simulink model "Generator_Testrig"  (R2025a)
settings: Solver=ode23t  StartTime=0.0  StopTime=15  MaxStep=0.01  RelTol=1e-5  EnableMultiTasking=on
PreLoadFcn:
  | load Generator_Test_DATA
PostLoadFcn:
  | warning off ne_sli:simulator:input:FilteredInputs
undefined symbols (not defined in the file or in its folder): radps2rpm
libraries: fl_lib x6, nesl_utility x4, Generator_Lib x3, Geartrain_Lib x1, simulink x1
Description:
  | Copyright 2009-2024 The MathWorks, Inc. MathWorks, Inc.
settings Model: Creator=smiller  LastModifiedBy=smiller
settings SolverCC: AlgebraicLoopSolver=TrustRegion
settings DataIOCC: LimitDataPoints=on  SaveFormat=Array  SignalLoggingSaveFormat=ModelDataLogs  ReturnWorkspaceOutputs=off
settings OptimizationCC: ReuseModelBlockBuffer=off  ExpressionDepthLimit=2147483647.0  LifeSpan=inf
settings DebuggingCC: UnderspecifiedInitializationDetection=Classic  MergeDetectMultiDrivingBlocksExec=none  SolverPrmCheckMsg=warning  FcnCallInpInsideContextMsg=warning  UnconnectedInputMsg=warning  UnconnectedOutputMsg=warning  UnconnectedLineMsg=warning  AllowSymbolicDim=off  StateNameClashWarn=warning  PregeneratedLibrarySubsystemCodeDiagnostic=none  SFUnexpectedBacktrackingDiag=warning  SFNoUnconditionalDefaultTransitionDiag=warning  SFExecutionAtInitializationDiag=none  ArithmeticOperatorsInVariantConditions=warning
settings HardwareCC: ProdBitPerPointer=32.0  ProdBitPerSizeT=32.0  ProdBitPerPtrDiffT=32.0  ProdLargestAtomicFloat=None  ProdIntDivRoundTo=Undefined  ProdEndianess=Unspecified  ProdWordSize=32.0  ProdHWDeviceType=32-bit Generic
settings ModelReferenceCC: EnableRefExpFcnMdlSchedulingChecks=on  PropagateSignalLabelsOutOfModel=off
settings SFSimCC: SimUseLocalCustomCode=off  CustomCodeUndefinedFunction=UseInterfaceOnly
settings RTWCC: RTWUseLocalCustomCode=off  GPUComputeCapability=3.5  DLArmComputeVersion=19.05
settings CodeAppCC: StateflowObjectComments=on
settings GRTTargetCC: TargetLangStandard=C89/C90 (ANSI)  CombineOutputUpdateFcns=off  GRTInterface=on
settings ConfigComp: CovMetricSettings=dw  CovSaveCumulativeToWorkspaceVar=on  CovSaveSingleToWorkspaceVar=on  CovExternalEMLEnable=off  CovSFcnEnable=off
settings SimscapeCC: SimscapeNormalizeSystem=off  SimscapeNominalValues="[{\"value\":\"10\",\"unit\":\"V\"},{\"value\":\"1\",\"unit\":\"A\"},{\"value\":\"10\",\"unit\":\"N*m\"},{\"value\":\"10\",\"unit\":\"bar\"},{\"value\":\"100\",\"unit\":\"kJ/kg\"},{\"value\":\"1\",\"unit\":\"kW\"},{\"value\":\"300\",\"unit\":\"K\"},{\"value\":\"100\",\"unit\":\"cm^3/s\"},{\"value\":\"1\",\"unit\":\"kN\"},{\"value\":\"1\",\"unit\":\"g/cm^3\"},{\"value\":\"1\",\"unit\":\"l\"},{\"value\":\"1\",\"unit\":\"cm^2\"},{\"value\":\"60\",\"unit\":\"Hz\"}]"  SimscapeLogType=all  SimscapeLogName=simlog_Generator_testrig  SimscapeLogLimitData=off

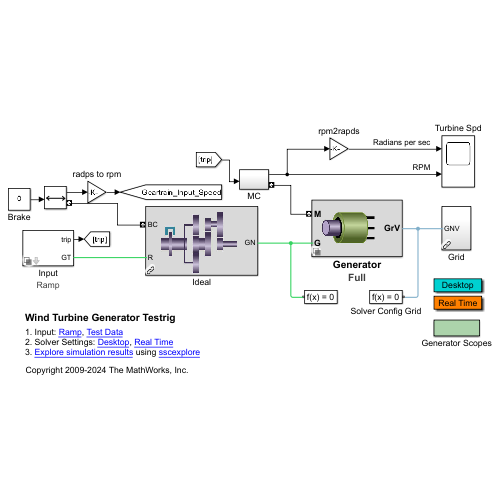
[thumbnail: Simulink's stored preview of the top-level diagram]
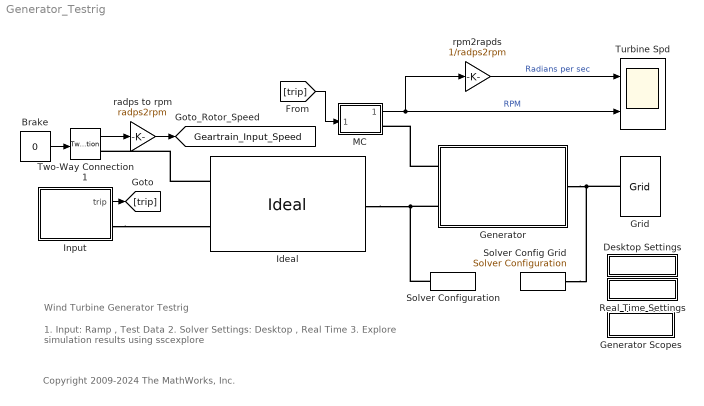
== system Generator_Testrig ==
  note: Copyright 2009-2024 The MathWorks, Inc.
  note: Wind Turbine Generator Testrig
  note: 1. Input: Ramp , Test Data
      | 2. Solver Settings: Desktop , Real Time
      | 3. Explore simulation results using sscexplore
  Brake : Constant  Value=0
  Desktop Settings : Subsystem
      settings: OpenFcn=|
      | set_param(bdroot,'Solver','ODE23t','MaxStep','0.01');
      | 
      | 
      | f    = Simulink.FindOptions('FollowLinks',0,'LookUnderMasks','none');
      | tvar_solverBlock = Simulink.findBlocks(bdroot, 'Name','Solver Configuration','SubClassName', 'solver',f);
      | 
      | for i=1:size(tvar_solverBlock,1)
      | 
      | set_param(tvar_solverBlock(i), 'UseLocalSolver','off','DoFixedCost','off');
      | end
      | 
      | clear tvar_solverBlock
      mask Display: disp('Desktop')
  Generator : Subsystem  Variant=on  VariantControlMode=label  LabelModeActiveChoice=Full
      settings: AttributesFormatString=%<ActiveVariant>
      mask Display:
      | blk = wind_turbine_activeVariantBlock(gcb);
      | eval(get_param(blk, 'MaskDisplay'));
  Generator Scopes : Subsystem  ReferencedSubsystem=Generator_Scopes
  Grid : Generator_Lib/Grid  SystemSampleTime=-1  VariantActivationTime=update diagram  EmptyChoice=off  PassThrough=off  PassThroughVariantControl=(default)  EmptyChoiceVariantControl=(default)  AllowFlexibleInterface=on  Latency=0  AutoFrameSizeCalculation=off
  Ideal : Geartrain_Lib/Ideal  SystemSampleTime=-1  VariantActivationTime=update diagram  EmptyChoice=off  PassThrough=off  PassThroughVariantControl=(default)  EmptyChoiceVariantControl=(default)  AllowFlexibleInterface=on  Latency=0  AutoFrameSizeCalculation=off
  Input : Subsystem  Variant=on  VariantControlMode=label  VariantControl=Ramp  LabelModeActiveChoice=Ramp  mask{popup_testrig_input=Ramp}
      mask prompts: popup_testrig_input "Testrig Input"
      mask init:
      | bh = gcb;
      | popupStr = get_param(bh,'popup_testrig_input');
      | if(startsWith(popupStr,'Test Data'))
      |     set_param(bh,'LabelModeActiveChoice','Data')
      | else
      |     set_param(bh,'LabelModeActiveChoice','Ramp')
      | end
      settings: AttributesFormatString=%<LabelModeActiveChoice>
      mask TypeOptions popup_testrig_input: Ramp | Test Data
      mask Display: disp(' ')
  MC : Subsystem
  Real Time Settings : Subsystem
      settings: OpenFcn=|
      | tvar_Nonlinear_Iterations = '3';
      | tvar_StepSize = '0.01';
      | %tvar_LocalSolver='NE_TRAPEZOIDAL_ADVANCER';
      | tvar_LocalSolver='NE_BACKWARD_EULER_ADVANCER';
      | set_param(bdroot,'Solver','ode1be','FixedStep','auto');
      | 
      | f    = Simulink.FindOptions('FollowLinks',0,'LookUnderMasks','none');
      | tvar_solverBlock = Simulink.findBlocks(bdroot,'Name','Solver Configuration','SubClassName', 'solver',f);
      | 
      | for i=1:size(tvar_solverBlock,1)
      |     set_param(tvar_solverBlock(i), 'UseLocalSolver','on','DoFixedCost','on','MaxNonlinIter',tvar_Nonlinear_Iterations,'LocalSolverChoice',tvar_LocalSolver,'LocalSolverSampleTime',tvar_StepSize);
      | end
      | clear tvar_Nonlinear_Iterations tvar_StepSize tvar_LocalSolver tvar_solverBlock
      mask Display: disp('Real Time')
  Solver Configuration : nesl_utility/Solver Configuration  PhysicalDomain=network_engine_domain  SubClassName=solver  LeftPortType=input  RightPortType=generic  Tones=[]  Harmonics=[]  SimulateNoise=off  Profile=off  UseLocalSampling=off  EnableSwitchedLinearOptims=on  FrequencyDomain=off  UseCCode=off  RelTol=0.001  AbsTol=1e-06  MinStep=1e-09  ToWorkspace=off  RevertToSquareIcSolve=off  NumHomotopyIterations=100  PhasorMode=off  PhasorModeNumHarmonics=1  ConsistencySolver=NEWTON_FTOL  IndexReductionMethod=DerivativeReplacement  DoDC=off  ResidualTolerance=1e-9  ConsistencyTolSource=GLOBAL  ConsistencyAbsTol=0.001  ConsistencyRelTol=0.001  ConsistencyTolFactor=0.001  UseLocalSolver=off  LocalSolverChoice=NE_BACKWARD_EULER_ADVANCER  ResolveIndetEquations=on  FunctionEvalNumThread=1  LocalSolverSampleTime=0.01  DoFixedCost=off  MaxNonlinIter=3  MaxModeIter=2  ComputeImpulses=off  ImpulseIterations=2  LinearAlgebra=Sparse  LinearAlgebraNumThread=0  EquationFormulation=NE_TIME_EF  DelaysMemoryBudget=1024  AutomaticFiltering=on  FilteringTimeConstant=0.001  PartitionStorageMethod=AS_NEEDED  PartitionMemoryBudget=1024  PartitionMethod=FAST  MultibodyUseLocalSolver=off  MultibodyLocalSolverChoice=ODE1  MultibodyLocalSolverSampleTime=0.001
  Solver Config Grid : nesl_utility/Solver Configuration  PhysicalDomain=network_engine_domain  SubClassName=solver  LeftPortType=input  RightPortType=generic  Tones=[]  Harmonics=[]  SimulateNoise=off  Profile=off  UseLocalSampling=off  EnableSwitchedLinearOptims=on  FrequencyDomain=off  UseCCode=off  RelTol=0.001  AbsTol=0.001  MinStep=1e-09  ToWorkspace=off  RevertToSquareIcSolve=off  NumHomotopyIterations=100  PhasorMode=off  PhasorModeNumHarmonics=1  ConsistencySolver=NEWTON_XTOL_AFTER_FTOL  IndexReductionMethod=None  DoDC=off  ResidualTolerance=1e-09  ConsistencyTolSource=GLOBAL  ConsistencyAbsTol=0.001  ConsistencyRelTol=0.001  ConsistencyTolFactor=1  UseLocalSolver=on  LocalSolverChoice=NE_BACKWARD_EULER_ADVANCER  ResolveIndetEquations=off  FunctionEvalNumThread=1  LocalSolverSampleTime=0.01  DoFixedCost=off  MaxNonlinIter=3  MaxModeIter=2  ComputeImpulses=off  ImpulseIterations=2  LinearAlgebra=auto  LinearAlgebraNumThread=0  EquationFormulation=NE_FREQUENCY_TIME_EF  DelaysMemoryBudget=1024  AutomaticFiltering=off  FilteringTimeConstant=0.001  PartitionStorageMethod=AS_NEEDED  PartitionMemoryBudget=1024  PartitionMethod=ROBUST  MultibodyUseLocalSolver=off  MultibodyLocalSolverChoice=ODE1  MultibodyLocalSolverSampleTime=0.001
  Turbine Spd : Scope  NumInputPorts=2
      settings: ActiveDisplayYMinimum=-20.51774  ActiveDisplayYMaximum=184.65966
  Two-Way Connection1 : TwoWayConnection
  radps to rpm : Gain  Gain=radps2rpm
  rpm2rapds : Gain  Gain=1/radps2rpm
  tag scope: Geartrain_Input_Speed=global
  wires:
  MC/1(Speed) -> rpm2rapds/1, Turbine Spd/2  "RPM"
  Two-Way Connection1/1 -> radps to rpm/1
  Brake/1 -> Two-Way Connection1/1
  radps to rpm/1 -> [Geartrain_Input_Speed]
  rpm2rapds/1 -> Turbine Spd/1  "Radians per sec"
  [trip] -> MC/1(Trip)
  Input/1(trip) -> [trip]
  connections:
  Ideal/RConn1 -- Generator/LConn2 -- Solver Configuration/RConn1
  Generator/LConn1 -- MC/RConn1
  Ideal/LConn1 -- Two-Way Connection1/RConn1
  Generator/RConn1 -- Grid/RConn1 -- Solver Config Grid/RConn1
  Input/RConn1 -- Ideal/LConn2

== system Generator_Testrig/Desktop Settings ==

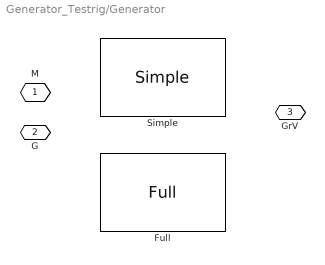
== system Generator_Testrig/Generator ==
  Full : Generator_Lib/Full  SystemSampleTime=-1  VariantControl=Full  VariantActivationTime=update diagram  EmptyChoice=off  PassThrough=off  PassThroughVariantControl=(default)  EmptyChoiceVariantControl=(default)  AllowFlexibleInterface=on  Latency=0  AutoFrameSizeCalculation=off
  Simple : Generator_Lib/Simple  SystemSampleTime=-1  VariantControl=Simple  VariantActivationTime=update diagram  AllowFlexibleInterface=on  Latency=0  AutoFrameSizeCalculation=off
  M : PMIOPort  Tag=PMCPort  Side=Left
  G : PMIOPort  Port=2  Side=Left
  GrV : PMIOPort  Port=3  Side=Right

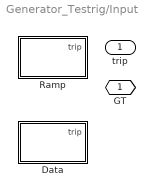
== system Generator_Testrig/Input ==
  Data : Subsystem  VariantControl=Data
  Ramp : Subsystem  VariantControl=Ramp  mask{start_speed=0, final_speed=14.3004, start_time=3, stop_time=10}
      mask prompts: start_speed "Start speed (rpm)"; final_speed "Final speed (rpm)"; start_time "Ramp start time"; stop_time "Ramp stop time"
  GT : PMIOPort  Side=Right
  trip : Outport

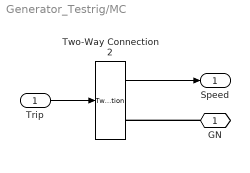
== system Generator_Testrig/MC ==
  Trip : Inport
  Two-Way Connection2 : TwoWayConnection
  GN : PMIOPort  Side=Right
  Speed : Outport  VectorParamsAs1DForOutWhenUnconnected=off
  wires:
  Two-Way Connection2/1 -> Speed/1
  Trip/1 -> Two-Way Connection2/1
  connections:
  GN/RConn1 -- Two-Way Connection2/RConn1

== system Generator_Testrig/Real Time Settings ==

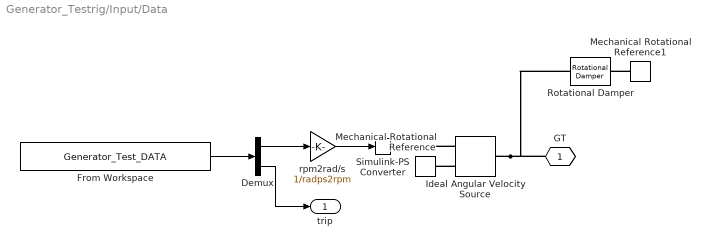
== system Generator_Testrig/Input/Data ==
  Demux : Demux  Outputs=2
  From Workspace : FromWorkspace  VariableName=Generator_Test_DATA
  Ideal Angular Velocity Source : fl_lib/Mechanical/Mechanical Sources/Ideal Angular Velocity Source
  Mechanical Rotational Reference : fl_lib/Mechanical/Rotational Elements/Mechanical Rotational Reference
  Mechanical Rotational Reference1 : fl_lib/Mechanical/Rotational Elements/Mechanical Rotational Reference
  Rotational Damper : fl_lib/Mechanical/Rotational Elements/Rotational Damper  D=0.001 N*m/(rad/s)  w_specify=off  w_priority=High  w=0 rad/s  w_nominal_specify=off  w_nominal_value=1  w_nominal_unit=rad/s  t_specify=off  t_priority=High  t=0 N*m  t_nominal_specify=off  t_nominal_value=1  t_nominal_unit=N*m
  Simulink-PS Converter : nesl_utility/Simulink-PS Converter  PhysicalDomain=network_engine_domain  SubClassName=ps_input  LeftPortType=input  RightPortType=output  PseudoPeriodic=off  Frequencies=[]  NoiseDistribution=none  NoiseParameters=[]  Unit=1  AffineConversion=off  FilteringAndDerivatives=zero  SimscapeFilterOrder=1  InputFilterTimeConstant=0.005  UdotUserProvided=0
  rpm2rad/s : Gain  Gain=1/radps2rpm
  GT : PMIOPort  Tag=PMCPort  Side=Right
  trip : Outport  VectorParamsAs1DForOutWhenUnconnected=off
  wires:
  rpm2rad/s/1 -> Simulink-PS Converter/1
  From Workspace/1 -> Demux/1
  Demux/1 -> rpm2rad/s/1
  Demux/2 -> trip/1
  connections:
  Ideal Angular Velocity Source/LConn1 -- GT/RConn1 -- Rotational Damper/LConn1
  Ideal Angular Velocity Source/RConn1 -- Simulink-PS Converter/RConn1
  Ideal Angular Velocity Source/RConn2 -- Mechanical Rotational Reference/LConn1
  Mechanical Rotational Reference1/LConn1 -- Rotational Damper/RConn1

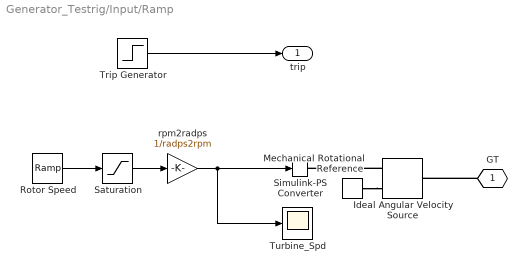
== system Generator_Testrig/Input/Ramp ==
  Ideal Angular Velocity Source : fl_lib/Mechanical/Mechanical Sources/Ideal Angular Velocity Source
  Mechanical Rotational Reference : fl_lib/Mechanical/Rotational Elements/Mechanical Rotational Reference
  Rotor Speed : simulink/Sources/Ramp  slope=(final_speed-start_speed)/(stop_time-start_time)  start=start_time  InitialOutput=start_speed
  Saturation : Saturate  UpperLimit=final_speed  LowerLimit=0
  Simulink-PS Converter : nesl_utility/Simulink-PS Converter  PhysicalDomain=network_engine_domain  SubClassName=ps_input  LeftPortType=input  RightPortType=output  PseudoPeriodic=off  Frequencies=[]  NoiseDistribution=none  NoiseParameters=[]  Unit=1  AffineConversion=off  FilteringAndDerivatives=filter  SimscapeFilterOrder=1  InputFilterTimeConstant=0.005  UdotUserProvided=1
  Trip Generator : Step  Time=10  Before=1  After=0  SampleTime=0
  Turbine_Spd : Scope
      settings: ActiveDisplayYMinimum=0  ActiveDisplayYMaximum=1.5
  rpm2radps : Gain  Gain=1/radps2rpm
  GT : PMIOPort  Tag=PMCPort  Side=Right
  trip : Outport
  wires:
  Rotor Speed/1 -> Saturation/1
  Saturation/1 -> rpm2radps/1
  rpm2radps/1 -> Turbine_Spd/1, Simulink-PS Converter/1
  Trip Generator/1 -> trip/1
  connections:
  GT/RConn1 -- Ideal Angular Velocity Source/LConn1
  Ideal Angular Velocity Source/RConn1 -- Simulink-PS Converter/RConn1
  Mechanical Rotational Reference/LConn1 -- Ideal Angular Velocity Source/RConn2
